simulink model "MotorModeloVideo"  (R2018a)
settings: Solver=VariableStepAuto  StartTime=0.0  StopTime=10.0  RelTol=1e-3
settings Model: Creator=Sergio  LastModifiedBy=Sergio

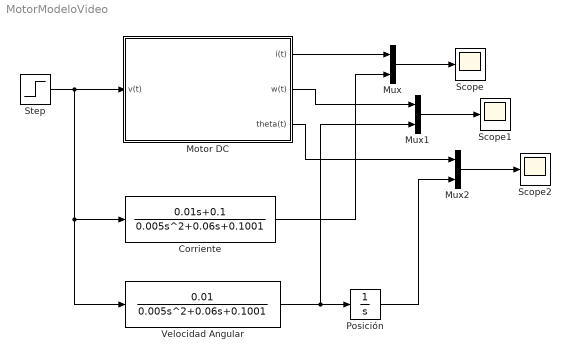
== system MotorModeloVideo ==
  Corriente : TransferFcn  Numerator=[0.01 0.1]  Denominator=[0.005 0.06 0.1001]
  Motor DC : Subsystem
  Mux : Mux  Inputs=2
  Mux1 : Mux  Inputs=2
  Mux2 : Mux  Inputs=2
  Posición : Integrator
  Scope : Scope
  Scope1 : Scope
  Scope2 : Scope
  Step : Step  Time=2  After=12  SampleTime=0
  Velocidad Angular : TransferFcn  Numerator=[0.01]  Denominator=[0.005 0.06 0.1001]
  wires:
  Velocidad Angular/1 -> Mux1/2, Posición/1
  Step/1 -> Corriente/1, Velocidad Angular/1, Motor DC/1(v(t))
  Motor DC/1(i(t)) -> Mux/1
  Mux/1 -> Scope/1
  Mux1/1 -> Scope1/1
  Mux2/1 -> Scope2/1
  Motor DC/2(w(t)) -> Mux1/1
  Motor DC/3(theta(t)) -> Mux2/1
  Posición/1 -> Mux2/2
  Corriente/1 -> Mux/2

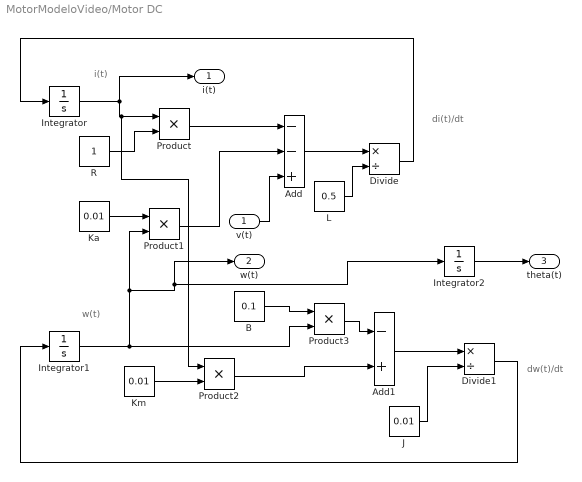
== system MotorModeloVideo/Motor DC ==
  note: i(t)
  note: w(t)
  note: di(t)/dt
  note: dw(t)/dt
  v(t) : Inport
  Add : Sum  Inputs=--+
  Add1 : Sum  Inputs=-+
  B : Constant  Value=0.1
  Divide : Product  Inputs=*/
  Divide1 : Product  Inputs=*/
  Integrator : Integrator
  Integrator1 : Integrator
  Integrator2 : Integrator
  J : Constant  Value=0.01
  Ka : Constant  Value=0.01
  Km : Constant  Value=0.01
  L : Constant  Value=0.5
  Product{,1..3} (4 alike) : Product
  R : Constant
  i(t) : Outport
  w(t) : Outport  Port=2
  theta(t) : Outport  Port=3
  wires:
  Divide/1 -> Integrator/1
  Integrator/1 -> i(t)/1, Product2/1, Product/1
  Integrator1/1 -> Product3/2, w(t)/1, Integrator2/1, Product1/2
  R/1 -> Product/2
  Add1/1 -> Divide1/1
  v(t)/1 -> Add/3
  Ka/1 -> Product1/1
  J/1 -> Divide1/2
  Product3/1 -> Add1/1
  Product1/1 -> Add/2
  Add/1 -> Divide/1
  Product/1 -> Add/1
  L/1 -> Divide/2
  Divide1/1 -> Integrator1/1
  Integrator2/1 -> theta(t)/1
  B/1 -> Product3/1
  Km/1 -> Product2/2
  Product2/1 -> Add1/2
